simulink model "ASM_Traffic_MultiCore"  (R2026a)
settings: Solver=ode1  StartTime=SIM.tstart.v  StopTime=SIM.tend.v  FixedStep=SIM.StepSize.v
PostLoadFcn:
  | if any(exist('dsrtsu_mdlpostloadfcn', 'file') ~= 0), dsrtsu_mdlpostloadfcn('Execute', bdroot); end
  | try, asm_mdl_postloadfcn(bdroot, 'UpdateModel', 3600); catch, disp(lasterr); end,
InitFcn:
  | , if any(exist('rtifpga_mdlclblib', 'file') ~= 0), rtifpga_mdlclblib('Init', bdroot); end,
  | , if any(exist('dsmpb_private', 'file') ~= 0), dsmpb_private('dsmpb_mdlclblib', 'Init', bdroot); end,
model workspace (MAT data in the model file):
  asmReferencePath = [0 0.01 0.02 0.03 0.04 0.05 0.06 0.07 0.08 0.09 0.1 0.11 ... (350007 elements, 50001x7)]
  roadBounds : Simulink.Parameter (value not decoded)
  safetyAxes : Simulink.Parameter (value not decoded)
undefined symbols (not defined in the file): _to_, a0b2, ASM_BrakeHydraulics_DemoSystems, ASM_VehicleDynamics_DemoSystems, b98103fe8ad365046cd0, BrakeCircuit, controllerConfig, CPT, Crankshaft, DiscIntNeverNeededParam, dsmsi, FinalDriveAssembly, MDL, ModeSignals, mu, Pos_BrakePedal_Maneuver, rad, RefSignals, roadFamilyData, roadFamilyId, s_to_rpm, SIM, SoftECU, Suspension, Tire, Transmission
libraries: ASM_Traffic_lib x135, simulink x98, ASM_Utils_lib x77, ASM_VehicleDynamics_lib x70, ASM_Environment_lib x22, dsmpblib x20, dsmsilib x15, MDLD_Utils_lib x10, ASM_BrakeHydraulics_lib x3, sl_discontinuities x2
(part 30 of 65)

== system ASM_Traffic_MultiCore/Environment/SignalInterface/ExternalOutports/Select_Outport_Signals ==
  ASMSignalBus : Inport
  Bus Creator1 : BusCreator  Inputs=8
  Bus Creator2 : BusCreator  Inputs=8
  Bus Creator3 : BusCreator  Inputs=6
  Bus Creator4 : BusCreator  Inputs=5
  Bus Selector : BusSelector  OutputSignals=Maneuver,Road,Traffic,GroundTruth,Sensors
  Bus Selector1 : BusSelector  OutputSignals=Parameter,SensorIndex,Info,SensorOutput,SensorTimeStamp,RadarEffects,CustomPoints,ObjectData
  Bus Selector2 : BusSelector  OutputSignals=Parameter,SensorIndex,Info,SensorOutput,SensorTimeStamp,RadarEffects,CustomPoints,ObjectData
  Bus Selector3 : BusSelector  OutputSignals=Parameters,SensorIndex,SensorStatus,SensorOutput,Info,ObjectData
  Bus Selector4 : BusSelector  OutputSignals=Collision_Sensor,TrafficSign_Sensor_Dyn,Object_Sensor_3D.Sensor_1_Front_Long,Object_Sensor_3D.Sensor_2_Front_Mid,Object_Sensor_2D.Sensor_1_Front
  Maneuver : Outport  VectorParamsAs1DForOutWhenUnconnected=off
  Road : Outport  Port=2  VectorParamsAs1DForOutWhenUnconnected=off
  Traffic : Outport  Port=3  VectorParamsAs1DForOutWhenUnconnected=off
  GroundTruth : Outport  Port=4  VectorParamsAs1DForOutWhenUnconnected=off
  Sensors : Outport  Port=5  VectorParamsAs1DForOutWhenUnconnected=off
  wires:
  Bus Selector3/6 -> Bus Creator3/6  "<ObjectData>"
  Bus Selector3/5 -> Bus Creator3/5  "<Info>"
  Bus Selector3/4 -> Bus Creator3/4  "<SensorOutput>"
  Bus Selector3/3 -> Bus Creator3/3  "<SensorStatus>"
  Bus Selector3/2 -> Bus Creator3/2  "<SensorIndex>"
  Bus Selector3/1 -> Bus Creator3/1  "<Parameters>"
  Bus Creator3/1 -> Bus Creator4/5  "Object_Sensor_2D_1"
  Bus Selector4/5 -> Bus Selector3/1  "<Sensor_1_Front>"
  Bus Selector4/4 -> Bus Selector2/1  "<Sensor_2_Front_Mid>"
  Bus Selector2/1 -> Bus Creator2/1  "<Parameter>"
  Bus Selector2/2 -> Bus Creator2/2  "<SensorIndex>"
  Bus Selector2/3 -> Bus Creator2/3  "<Info>"
  Bus Selector2/4 -> Bus Creator2/4  "<SensorOutput>"
  Bus Selector2/5 -> Bus Creator2/5  "<SensorTimeStamp>"
  Bus Selector2/6 -> Bus Creator2/6  "<RadarEffects>"
  Bus Selector2/7 -> Bus Creator2/7  "<CustomPoints>"
  Bus Selector2/8 -> Bus Creator2/8  "<ObjectData>"
  Bus Creator2/1 -> Bus Creator4/4  "Object_Sensor_3D_2"
  Bus Creator1/1 -> Bus Creator4/3  "Object_Sensor_3D_1"
  Bus Selector1/8 -> Bus Creator1/8  "<ObjectData>"
  Bus Selector1/7 -> Bus Creator1/7  "<CustomPoints>"
  Bus Selector1/6 -> Bus Creator1/6  "<RadarEffects>"
  Bus Selector1/5 -> Bus Creator1/5  "<SensorTimeStamp>"
  Bus Selector1/4 -> Bus Creator1/4  "<SensorOutput>"
  Bus Selector1/3 -> Bus Creator1/3  "<Info>"
  Bus Selector1/2 -> Bus Creator1/2  "<SensorIndex>"
  Bus Selector1/1 -> Bus Creator1/1  "<Parameter>"
  Bus Selector4/3 -> Bus Selector1/1  "<Sensor_1_Front_Long>"
  Bus Selector4/2 -> Bus Creator4/2  "<TrafficSign_Sensor_Dyn>"
  Bus Selector/2 -> Road/1  "<Road>"
  Bus Selector/3 -> Traffic/1  "<Traffic>"
  Bus Selector/1 -> Maneuver/1  "<Maneuver>"
  ASMSignalBus/1 -> Bus Selector/1
  Bus Selector/4 -> GroundTruth/1  "<GroundTruth>"
  Bus Selector/5 -> Bus Selector4/1  "<Sensors>"
  Bus Selector4/1 -> Bus Creator4/1  "<Collision_Sensor>"
  Bus Creator4/1 -> Sensors/1  "Sensors"

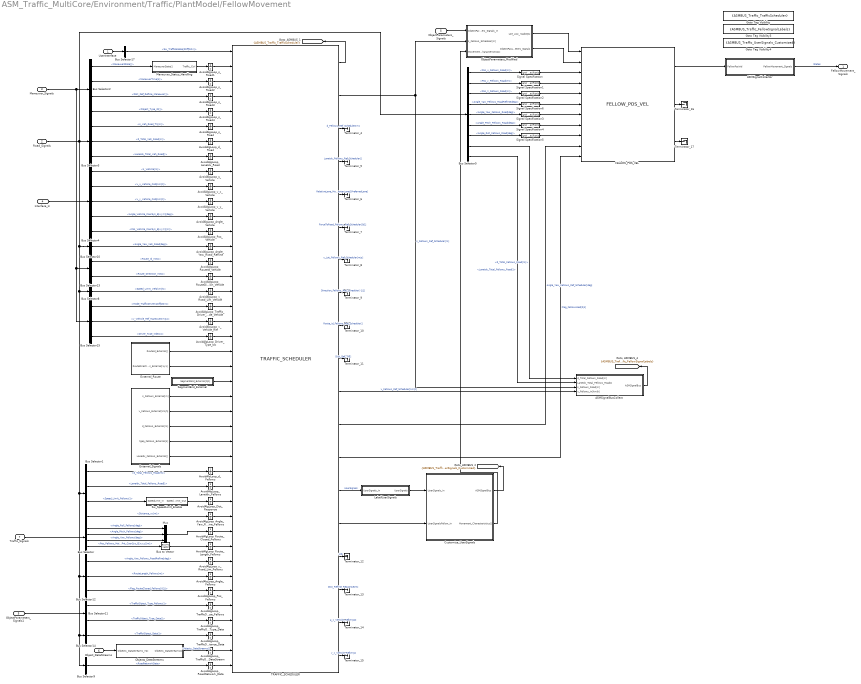
== system ASM_Traffic_MultiCore/Environment/Traffic/PlantModel/FellowMovement ==
  UserInterface : Inport
  Road_Signals : Inport  Port=2
  Maneuver_Signals : Inport  Port=3
  Interface_In : Inport  Port=4
  ObjectParameters_Signals : Inport  Port=5
  Object_DataStreams : Inport  Port=6
  Traffic_Signals : Inport  Port=7
  ASMSignalBusCollect : Subsystem
  ASMSignalCollector : Subsystem
  AvoidAlgLoop_Angle_Fellows : UnitDelay  SampleTime=-1
  AvoidAlgLoop_Angle_Vehicle : UnitDelay  SampleTime=-1
  AvoidAlgLoop_Angle_Yaw_RoadRefline_Fellows : UnitDelay  SampleTime=-1
  AvoidAlgLoop_Angle_Yaw_Road_Refline : UnitDelay  SampleTime=-1
  AvoidAlgLoop_Dist_Response : UnitDelay  SampleTime=-1
  AvoidAlgLoop_Driver_Type_Idx : UnitDelay  SampleTime=-1
  AvoidAlgLoop_LaneIdx_Fellows : UnitDelay  SampleTime=-1
  AvoidAlgLoop_LaneIdx_Road : UnitDelay  SampleTime=-1
  AvoidAlgLoop_Pos_Fellows : UnitDelay  SampleTime=-1
  AvoidAlgLoop_Pos_Vehicle : UnitDelay  SampleTime=-1
  AvoidAlgLoop_RoadNetwork_Data : UnitDelay  SampleTime=-1
  AvoidAlgLoop_RouteDirection_Vehicle : UnitDelay  SampleTime=-1
  AvoidAlgLoop_RouteId_Vehicle : UnitDelay  SampleTime=-1
  AvoidAlgLoop_Route_Closed_Fellows : UnitDelay  SampleTime=-1
  AvoidAlgLoop_Route_Length_Fellows : UnitDelay  SampleTime=-1
  AvoidAlgLoop_TrafficObject_DataStream : UnitDelay  SampleTime=-1
  AvoidAlgLoop_TrafficObject_Instance_Data : UnitDelay  SampleTime=-1
  AvoidAlgLoop_TrafficObject_Type_Data : UnitDelay  SampleTime=-1
  AvoidAlgLoop_TrafficObject_Type_Fellows : UnitDelay  SampleTime=-1
  AvoidAlgLoop_Traffic_Driver_Mode_Vehicle : UnitDelay  SampleTime=-1
  AvoidAlgLoop_d_Fellows : UnitDelay  SampleTime=-1
  AvoidAlgLoop_d_Road : UnitDelay  SampleTime=-1
  AvoidAlgLoop_s_Road{,1..4} (5 alike) : UnitDelay  SampleTime=-1
  AvoidAlgLoop_s_Vehicle : UnitDelay  SampleTime=-1
  AvoidAlgLoop_v_Road_Lim_Fellows : UnitDelay  SampleTime=-1
  AvoidAlgLoop_v_Road_Lim_Vehicle : UnitDelay  SampleTime=-1
  AvoidAlgLoop_v_Vehicle_Ref : UnitDelay  SampleTime=-1
  AvoidAlgLoop_v_x_Vehicle : UnitDelay  SampleTime=-1
  AvoidAlgLoop_v_y_Vehicle : UnitDelay  SampleTime=-1
  Bus Selector : BusSelector  OutputSignals=Plant.Traffic_Signals_toEnvironment.Angle_Fellows[x;y;z][deg].Angle_Roll_Fellows[deg],Plant.Traffic_Signals_toEnvironment.Angle_Fellows[x;y;z][deg].Angle_Pitch_Fellows[deg],Plant.Traffic_Signals_toEnvironment.Angle_Fellows[x;y;z][deg].Angle_Yaw_Fellows[deg],Plant.Traffic_Signals_toEnvironment.Pos_Fellows_MainPnt_CoorSys_E[x;y;z][m]
  Bus Selector1 : BusSelector  OutputSignals=Plant.Road_TrafficFellows.d_Total_Fellows_Road[m],Plant.Road_TrafficFellows.LaneIdx_Total_Fellows_Road[],Plant.Road_TrafficFellows.Speed_Limit_Fellows[],Plant.Road_TrafficFellows.Dist_Response_Traffic.Distance_xy[m]
  Bus Selector10 : BusSelector  OutputSignals=Plant.Road_ASMVeh.Angle_Yaw_Veh_Road[deg]
  Bus Selector11 : BusSelector  OutputSignals=FellowParameters.TrafficObject_Type_Fellows[],TrafficObjects.TrafficObject_Type_Data[]
  Bus Selector12 : BusSelector  OutputSignals=Plant.Road_TrafficFellows.Angle_Yaw_Fellows_RoadRefline[deg],Plant.Road_TrafficFellows.RouteLength_Fellows[m],Plant.Road_TrafficFellows.Flag_RouteClosed_Fellows[0|1]
  Bus Selector13 : BusSelector  OutputSignals=Plant.ManeuverScheduler.InitialVehStates.Route_Id_Init[],Plant.ManeuverScheduler.InitialVehStates.Route_Direction_Init[]
  Bus Selector14 : BusSelector  OutputSignals=Plant.TrafficObject_Data[]
  Bus Selector15 : BusSelector  OutputSignals=Plant.ManeuverScheduler.ModeSignals.Mode_TrafficDriver[1Off|2On],Plant.ManeuverScheduler.RefSignals.v_Vehicle_Ref_Maneuver[m|s],Plant.ManeuverScheduler.Parameters.Driver_Type_Index[]
  Bus Selector17 : BusSelector  OutputSignals=Sw_TrafficEnable[0Off|1On]
  Bus Selector2 : BusSelector  OutputSignals=Plant.ManeuverScheduler.Info.ManeuverState[],Plant.ManeuverScheduler.Info.ManeuverTime[s],Plant.ManeuverScheduler.RefSignals.Dist_Def_Refline_Maneuver[],Plant.ManeuverScheduler.Parameters.Object_Type_ID[]
  Bus Selector3 : BusSelector  OutputSignals=Plant.Road_ASMVeh.s_Veh_Road_Trj[m],Plant.Road_ASMVeh.d_Total_Veh_Road[m],Plant.Road_ASMVeh.LaneIdx_Total_Veh_Road[]
  Bus Selector4 : BusSelector  OutputSignals=ExternalModel.s_Vehicle[m],ExternalModel.v_x_Vehicle_CoG[km|h],ExternalModel.v_y_Vehicle_CoG[km|h],ExternalModel.Angle_Vehicle_CoorSys_E[x;y;z][deg],ExternalModel.Pos_Vehicle_CoorSys_E[x;y;z][m]
  Bus Selector5 : BusSelector  OutputSignals=Plant.Road_TrafficFellows.Pos_x_Fellows_Road[m],Plant.Road_TrafficFellows.Pos_y_Fellows_Road[m],Plant.Road_TrafficFellows.Pos_z_Fellows_Road[m],Plant.Road_TrafficFellows.Angle_Yaw_Fellows_RoadRefline[deg],Plant.Road_TrafficFellows.Angle_Yaw_Fellows_Road[deg],Plant.Road_TrafficFellows.Angle_Pitch_Fellows_Road[deg],Plant.Road_TrafficFellows.Angle_Roll_Fellows_Road[deg],Plant.Road_TrafficFellows.d_Total_Fellows_Road[m],Plant.Road_TrafficFellows.LaneIdx_Total_Fellows_Road[]
  Bus Selector8 : BusSelector  OutputSignals=Plant.Road_Info.Speed_Limit_Veh[km|h]
  Bus Selector9 : BusSelector  OutputSignals=Plant.Road_Info.Trf_Driver_Data.RoadNetworkData
  Bus to Vector : BusToVector
  Customize_UserSignals : Subsystem
  External_Route : Subsystem
  External_Signals : Subsystem
  FELLOW_POS_VEL : ASM_Traffic_lib/Movement/FELLOW_POS_VEL  StepSize=SIM.StepSize  ASMProperties=struct('Name','FELLOW_POS_VEL','Version','2.0','Library','ASM_Traffic_lib')  ASMInstanceName=fellow_pos_vel  ASMInstanceID=1
  Goto Tag Visibility : GotoTagVisibility  GotoTag=ASMBUS_Traffic_TrafficScheduler
  Goto Tag Visibility3 : GotoTagVisibility  GotoTag=ASMBUS_Traffic_FellowSignalLabels
  Goto Tag Visibility4 : GotoTagVisibility  GotoTag=ASMBUS_Traffic_UserSignals_Customized
  LabelUserSignals : Subsystem
  Maneuver_Status_Handling : Subsystem
  Mux : Mux  Inputs=3
  ObjectParameters_Modified : Subsystem
  ObjectParameters_Signals1 : InportShadow  Port=5
  Objects_DataStreams : Subsystem
  SegmentEnd_External : Subsystem
  Signal Specification{,1..6} (7 alike) : SignalSpecification  Dimensions=MDL.Traffic.MaxNumFellows.v
  Sw_SpeedLimit_Enable : Subsystem
  TRAFFIC_SCHEDULER : ASM_Traffic_lib/Movement/TRAFFIC_SCHEDULER  Tag=ASM_SUBCOMPONENT  TrafficVector=MDL.Traffic.TrafficScheduler.Scenario  MaxNumFellows=MDL.Traffic.MaxNumFellows  MaxNumFDUserSignals=MDL.Traffic.MaxNumFDUserSignals  MaxNumUserSignals=MDL.Traffic.MaxNumUserSignals  StepSize=SIM.StepSize  ASMProperties=struct('Name','TRAFFIC_SCHEDULER','Version','23.0','Library','ASM_Traffic_lib')  ASMInstanceName=traffic_scheduler  ASMInstanceID=1
  Terminator_{4..17} (14 alike) : Terminator
  FellowMovement_Signals : Outport  VectorParamsAs1DForOutWhenUnconnected=off
  tag scope: ASMBUS_Traffic_FellowSignalLabels=scoped, ASMBUS_Traffic_TrafficScheduler=scoped, ASMBUS_Traffic_UserSignals_Customized=scoped
  wires:
  ObjectParameters_Modified/2(ObjectParameters_Signals) -> FELLOW_POS_VEL/2
  FELLOW_POS_VEL/1 -> ASMSignalCollector/1(FellowPosVel)
  TRAFFIC_SCHEDULER/19 -> Terminator_15/1  "v_x_Vehicle_Ref[m|s]"
  TRAFFIC_SCHEDULER/18 -> Terminator_14/1  "a_x_Vehicle_Ref[m|s2]"
  TRAFFIC_SCHEDULER/17 -> Terminator_13/1  "Dist_Refline_Response[m]"
  TRAFFIC_SCHEDULER/16 -> Terminator_12/1  "Info"
  TRAFFIC_SCHEDULER/10 -> Terminator_11/1  "Dist_Def_Trf[]"
  TRAFFIC_SCHEDULER/9 -> Terminator_10/1  "Route_Id_Fellows_Ref_Scheduler[]"
  TRAFFIC_SCHEDULER/8 -> Terminator_9/1  "Direction_Fellows_Ref_Scheduler[-1|1]"
  TRAFFIC_SCHEDULER/7 -> Terminator_8/1  "v_Lat_Fellows_Ref_Scheduler[m|s]"
  TRAFFIC_SCHEDULER/6 -> Terminator_7/1  "ForceToRoad_Fellows_Ref_Scheduler[0|1]"
  TRAFFIC_SCHEDULER/5 -> Terminator_6/1  "RelativeLane_Mode_Fellows[0CenterLane|1PreferredLane]"
  TRAFFIC_SCHEDULER/4 -> Terminator_5/1  "LaneIdx_Fellows_Ref_Scheduler[]"
  TRAFFIC_SCHEDULER/3 -> Terminator_4/1  "d_Fellows_Ref_Scheduler[m]"
  Customize_UserSignals/2(Movement_Characteristics[]) -> ObjectParameters_Modified/3(Movement_Characteristics[])
  ASMSignalCollector/1(FellowMovement_Signals) -> FellowMovement_Signals/1  "States"
  Object_DataStreams/1 -> Objects_DataStreams/1(Objects_DataStreams_In[])
  Bus Selector17/1 -> TRAFFIC_SCHEDULER/1  "<Sw_TrafficEnable[0Off|1On]>"
  UserInterface/1 -> Bus Selector17/1
  TRAFFIC_SCHEDULER/11 -> ASMSignalBusCollect/4(v_Fellows_In[km|h])  "v_Fellows_Ref_Scheduler[km|h]"
  TRAFFIC_SCHEDULER/12 -> FELLOW_POS_VEL/10  "Angle_Yaw_Fellows_Ref_Scheduler[deg]"
  TRAFFIC_SCHEDULER/13 -> FELLOW_POS_VEL/11  "Flag_FellowUsed[0|1]"
  TRAFFIC_SCHEDULER/14 -> LabelUserSignals/1(UserSignals_In)  "UserSignals"
  TRAFFIC_SCHEDULER/15 -> Customize_UserSignals/2(UserSignalsFellow_In)
  Bus Selector12/3 -> AvoidAlgLoop_Pos_Fellows/1  "<Flag_RouteClosed_Fellows[0|1]>"
  Bus Selector12/2 -> AvoidAlgLoop_Angle_Fellows/1  "<RouteLength_Fellows[m]>"
  Bus Selector12/1 -> AvoidAlgLoop_v_Road_Lim_Fellows/1  "<Angle_Yaw_Fellows_RoadRefline[deg]>"
  Bus Selector1/3 -> Sw_SpeedLimit_Enable/1(SpeedLimit_In)  "<Speed_Limit_Fellows[]>"
  Sw_SpeedLimit_Enable/1(SpeedLimit_Out) -> AvoidAlgLoop_Dist_Response/1
  AvoidAlgLoop_TrafficObject_DataStream/1 -> TRAFFIC_SCHEDULER/41
  Objects_DataStreams/1(Objects_DataStreams[]) -> AvoidAlgLoop_TrafficObject_DataStream/1  "Objects_DataStreams[]"
  AvoidAlgLoop_RoadNetwork_Data/1 -> TRAFFIC_SCHEDULER/42
  Bus Selector8/1 -> AvoidAlgLoop_v_Road_Lim_Vehicle/1  "<Speed_Limit_Veh[km|h]>"
  Bus Selector4/5 -> AvoidAlgLoop_Pos_Vehicle/1  "<Pos_Vehicle_CoorSys_E[x;y;z][m]>"
  Bus Selector4/4 -> AvoidAlgLoop_Angle_Vehicle/1  "<Angle_Vehicle_CoorSys_E[x;y;z][deg]>"
  AvoidAlgLoop_Angle_Vehicle/1 -> TRAFFIC_SCHEDULER/12
  AvoidAlgLoop_Pos_Fellows/1 -> TRAFFIC_SCHEDULER/37
  AvoidAlgLoop_v_Road_Lim_Vehicle/1 -> TRAFFIC_SCHEDULER/17
  Bus Selector15/3 -> AvoidAlgLoop_Driver_Type_Idx/1  "<Driver_Type_Index[]>"
  Bus Selector15/1 -> AvoidAlgLoop_Traffic_Driver_Mode_Vehicle/1  "<Mode_TrafficDriver[1Off|2On]>"
  AvoidAlgLoop_Traffic_Driver_Mode_Vehicle/1 -> TRAFFIC_SCHEDULER/18
  AvoidAlgLoop_Driver_Type_Idx/1 -> TRAFFIC_SCHEDULER/20
  AvoidAlgLoop_v_Vehicle_Ref/1 -> TRAFFIC_SCHEDULER/19
  Bus Selector15/2 -> AvoidAlgLoop_v_Vehicle_Ref/1  "<v_Vehicle_Ref_Maneuver[m|s]>"
  AvoidAlgLoop_v_y_Vehicle/1 -> TRAFFIC_SCHEDULER/11
  AvoidAlgLoop_Pos_Vehicle/1 -> TRAFFIC_SCHEDULER/13
  Maneuver_Signals/1 -> Bus Selector13/1, Bus Selector15/1, Bus Selector2/1
  AvoidAlgLoop_LaneIdx_Fellows/1 -> TRAFFIC_SCHEDULER/30
  AvoidAlgLoop_v_Road_Lim_Fellows/1 -> TRAFFIC_SCHEDULER/35
  AvoidAlgLoop_Angle_Yaw_RoadRefline_Fellows/1 -> TRAFFIC_SCHEDULER/32
  Bus Selector14/1 -> AvoidAlgLoop_TrafficObject_Instance_Data/1  "<TrafficObject_Data[]>"
  Bus Selector9/1 -> AvoidAlgLoop_RoadNetwork_Data/1  "<RoadNetworkData>"
  AvoidAlgLoop_s_Road3/1 -> TRAFFIC_SCHEDULER/4
  AvoidAlgLoop_s_Road/1 -> TRAFFIC_SCHEDULER/6
  AvoidAlgLoop_RouteDirection_Vehicle/1 -> TRAFFIC_SCHEDULER/16
  TRAFFIC_SCHEDULER/1 -> [ASMBUS_Traffic_TrafficScheduler]
  AvoidAlgLoop_s_Road2/1 -> TRAFFIC_SCHEDULER/3
  External_Signals/3(d_Fellows_External[m]) -> TRAFFIC_SCHEDULER/26
  External_Signals/1(s_Fellows_External[m]) -> TRAFFIC_SCHEDULER/24
  AvoidAlgLoop_TrafficObject_Type_Data/1 -> TRAFFIC_SCHEDULER/39
  AvoidAlgLoop_v_x_Vehicle/1 -> TRAFFIC_SCHEDULER/10
  AvoidAlgLoop_TrafficObject_Type_Fellows/1 -> TRAFFIC_SCHEDULER/38
  External_Signals/2(v_Fellows_External[km|h]) -> TRAFFIC_SCHEDULER/25
  AvoidAlgLoop_s_Road4/1 -> TRAFFIC_SCHEDULER/5
  Bus Selector13/1 -> AvoidAlgLoop_RouteId_Vehicle/1  "<Route_Id_Init[]>"
  AvoidAlgLoop_Angle_Fellows/1 -> TRAFFIC_SCHEDULER/36
  AvoidAlgLoop_s_Vehicle/1 -> TRAFFIC_SCHEDULER/9
  AvoidAlgLoop_d_Fellows/1 -> TRAFFIC_SCHEDULER/29
  Bus Selector4/1 -> AvoidAlgLoop_s_Vehicle/1  "<s_Vehicle[m]>"
  Bus Selector11/1 -> AvoidAlgLoop_TrafficObject_Type_Fellows/1  "<TrafficObject_Type_Fellows[]>"
  AvoidAlgLoop_TrafficObject_Instance_Data/1 -> TRAFFIC_SCHEDULER/40
  Bus Selector2/4 -> AvoidAlgLoop_s_Road4/1  "<Object_Type_ID[]>"
  Bus Selector3/3 -> AvoidAlgLoop_LaneIdx_Road/1  "<LaneIdx_Total_Veh_Road[]>"
  Interface_In/1 -> Bus Selector4/1
  Bus Selector3/1 -> AvoidAlgLoop_s_Road/1  "<s_Veh_Road_Trj[m]>"
  Bus Selector4/3 -> AvoidAlgLoop_v_y_Vehicle/1  "<v_y_Vehicle_CoG[km|h]>"
  Maneuver_Status_Handling/1(Traffic_Ctrl) -> AvoidAlgLoop_s_Road1/1
  Bus Selector1/1 -> AvoidAlgLoop_d_Fellows/1  "<d_Total_Fellows_Road[m]>"
  Bus Selector1/2 -> AvoidAlgLoop_LaneIdx_Fellows/1  "<LaneIdx_Total_Fellows_Road[]>"
  Bus Selector3/2 -> AvoidAlgLoop_d_Road/1  "<d_Total_Veh_Road[m]>"
  Bus Selector2/1 -> Maneuver_Status_Handling/1(ManeuverState[])  "<ManeuverState[]>"
  Bus Selector4/2 -> AvoidAlgLoop_v_x_Vehicle/1  "<v_x_Vehicle_CoG[km|h]>"
  TRAFFIC_SCHEDULER/2 -> ObjectParameters_Modified/2(s_Fellows_Scheduler[m]), ASMSignalBusCollect/3(s_Fellows_Road[m])  "s_Fellows_Ref_Scheduler[m]"
  AvoidAlgLoop_LaneIdx_Road/1 -> TRAFFIC_SCHEDULER/8
  Bus Selector2/2 -> AvoidAlgLoop_s_Road2/1  "<ManeuverTime[s]>"
  AvoidAlgLoop_Dist_Response/1 -> TRAFFIC_SCHEDULER/31
  LabelUserSignals/1(UserSignals) -> Customize_UserSignals/1(UserSignals_In)
  Road_Signals/1 -> Bus Selector3/1, Bus Selector10/1, Bus Selector1/1, Bus Selector12/1, Bus Selector14/1, Bus Selector9/1, Bus Selector8/1, Bus Selector5/1
  Bus Selector2/3 -> AvoidAlgLoop_s_Road3/1  "<Dist_Def_Refline_Maneuver[]>"
  AvoidAlgLoop_d_Road/1 -> TRAFFIC_SCHEDULER/7
  ObjectParameters_Signals1/1 -> Bus Selector11/1
  Bus Selector10/1 -> AvoidAlgLoop_Angle_Yaw_Road_Refline/1  "<Angle_Yaw_Veh_Road[deg]>"
  AvoidAlgLoop_RouteId_Vehicle/1 -> TRAFFIC_SCHEDULER/15
  AvoidAlgLoop_s_Road1/1 -> TRAFFIC_SCHEDULER/2
  External_Route/1(RouteId_External[]) -> TRAFFIC_SCHEDULER/21
  Bus Selector11/2 -> AvoidAlgLoop_TrafficObject_Type_Data/1  "<TrafficObject_Type_Data[]>"
  External_Signals/4(tgap_Fellows_External[s]) -> TRAFFIC_SCHEDULER/27
  SegmentEnd_External/1(SegmentEnd_External[0|1]) -> TRAFFIC_SCHEDULER/23
  AvoidAlgLoop_Angle_Yaw_Road_Refline/1 -> TRAFFIC_SCHEDULER/14
  Bus Selector1/4 -> AvoidAlgLoop_Angle_Yaw_RoadRefline_Fellows/1  "<Distance_xy[m]>"
  Bus Selector13/2 -> AvoidAlgLoop_RouteDirection_Vehicle/1  "<Route_Direction_Init[]>"
  External_Signals/5(LaneIdx_Fellows_External[]) -> TRAFFIC_SCHEDULER/28
  External_Route/2(RouteDirection_External[1|-1]) -> TRAFFIC_SCHEDULER/22
  ASMSignalBusCollect/1(ASMSignalBus) -> [ASMBUS_Traffic_FellowSignalLabels]
  Bus Selector5/9 -> ASMSignalBusCollect/2(LaneIdx_Total_Fellows_Road[])  "<LaneIdx_Total_Fellows_Road[]>"
  Bus Selector5/8 -> ASMSignalBusCollect/1(d_Total_Fellows_Road[m])  "<d_Total_Fellows_Road[m]>"
  Customize_UserSignals/1(ASMSignalBus) -> [ASMBUS_Traffic_UserSignals_Customized]
  ObjectParameters_Signals/1 -> ObjectParameters_Modified/1(ObjectParameters_Signals_In)
  Bus Selector5/7 -> Signal Specification5/1  "<Angle_Roll_Fellows_Road[deg]>"
  Bus Selector5/6 -> Signal Specification4/1  "<Angle_Pitch_Fellows_Road[deg]>"
  Bus Selector5/5 -> Signal Specification3/1  "<Angle_Yaw_Fellows_Road[deg]>"
  Bus Selector5/3 -> Signal Specification2/1  "<Pos_z_Fellows_Road[m]>"
  Bus Selector5/2 -> Signal Specification1/1  "<Pos_y_Fellows_Road[m]>"
  Bus Selector5/1 -> Signal Specification/1  "<Pos_x_Fellows_Road[m]>"
  Signal Specification/1 -> FELLOW_POS_VEL/3
  Signal Specification1/1 -> FELLOW_POS_VEL/4
  Signal Specification2/1 -> FELLOW_POS_VEL/5
  Signal Specification4/1 -> FELLOW_POS_VEL/8
  Signal Specification5/1 -> FELLOW_POS_VEL/9
  FELLOW_POS_VEL/2 -> Terminator_16/1
  FELLOW_POS_VEL/3 -> Terminator_17/1
  Traffic_Signals/1 -> Bus Selector/1
  Bus Selector/4 -> Bus to Vector/1  "<Pos_Fellows_MainPnt_CoorSys_E[x;y;z][m]>"
  Bus to Vector/1 -> AvoidAlgLoop_Route_Length_Fellows/1
  Mux/1 -> AvoidAlgLoop_Route_Closed_Fellows/1
  Bus Selector/1 -> Mux/1  "<Angle_Roll_Fellows[deg]>"
  Bus Selector/2 -> Mux/2  "<Angle_Pitch_Fellows[deg]>"
  Bus Selector/3 -> Mux/3  "<Angle_Yaw_Fellows[deg]>"
  AvoidAlgLoop_Route_Closed_Fellows/1 -> TRAFFIC_SCHEDULER/33
  AvoidAlgLoop_Route_Length_Fellows/1 -> TRAFFIC_SCHEDULER/34
  Bus Selector5/4 -> Signal Specification6/1  "<Angle_Yaw_Fellows_RoadRefline[deg]>"
  Signal Specification3/1 -> FELLOW_POS_VEL/7
  Signal Specification6/1 -> FELLOW_POS_VEL/6
  ObjectParameters_Modified/1(use_yaw_road[0|1]) -> FELLOW_POS_VEL/1

== system ASM_Traffic_MultiCore/Environment/Traffic/PlantModel/Merge_Signals_toEnvironment ==
  Traffic_Signals : Inport
  GroundTruth_Interface : Inport  Port=2
  Bus Creator : BusCreator  Inputs=26
  Bus Selector : BusSelector  OutputSignals=TrafficScheduler
  Bus Selector1 : BusSelector  OutputSignals=Plant.Control
  Bus Selector2 : BusSelector  OutputSignals=s_Fellows_Ref_Scheduler[m],d_Fellows_Ref_Scheduler[m],v_Fellows_Ref_Scheduler[km|h],LaneIdx_Fellows_Ref_Scheduler[],RelativeLane_Mode_Fellows[0CenterLane|1PreferredLane],ForceToRoad_Fellows_Ref_Scheduler[0|1],v_Lat_Fellows_Ref_Scheduler[m|s],Direction_Fellows_Ref_Scheduler[-1|1],Route_Id_Fellows_Ref_Scheduler[],Dist_Def_Trf[],Flag_FellowUsed[0|1],a_x_Vehicle_Ref[m|s2],Dist_Refline_Response[m],Info,a_Fellows_Ref_Scheduler[m|s2],UserSignals_Fellows[]
  Bus Selector3 : BusSelector  OutputSignals=FellowPositions
  Bus Selector4 : BusSelector  OutputSignals=FellowSignalLabels
  Bus Selector5 : BusSelector  OutputSignals=d_Total_Fellows[m],LaneIdx_Total_Fellows[],v_Fellows[km|h]
  Bus Selector6 : BusSelector  OutputSignals=Pos_Fellows_MainPnt_CoorSys_E[x;y;z][m],Angle_Fellows[x;y;z][deg],Angle_Fellows[x;y;z][deg].Angle_Wheel_Fellows[deg]
  Bus Selector7 : BusSelector  OutputSignals=FellowVelocities
  Bus Selector8 : BusSelector  OutputSignals=v_Fellows[x;y;z][km|h],w_Fellows[x;y;z][deg|s]
  Bus Selector9 : BusSelector  OutputSignals=UserSignals_Customized
  avoid_incomplete_trace2source : Subsystem
  Signals_toEnvironment : Outport  VectorParamsAs1DForOutWhenUnconnected=off
  wires:
  avoid_incomplete_trace2source/1(Out1) -> Bus Creator/26  "Control"
  Bus Selector1/1 -> avoid_incomplete_trace2source/1(In1)  "<Control>"
  Bus Selector9/1 -> Bus Creator/25  "<UserSignals_Customized>"
  Bus Selector8/2 -> Bus Creator/24  "<w_Fellows[x;y;z][deg|s]>"
  Bus Selector8/1 -> Bus Creator/23  "<v_Fellows[x;y;z][km|h]>"
  Bus Selector6/3 -> Bus Creator/22  "<Angle_Wheel_Fellows[deg]>"
  Bus Selector6/2 -> Bus Creator/21  "<Angle_Fellows[x;y;z][deg]>"
  Bus Selector6/1 -> Bus Creator/20  "<Pos_Fellows_MainPnt_CoorSys_E[x;y;z][m]>"
  Bus Selector5/3 -> Bus Creator/19  "<v_Fellows[km|h]>"
  Bus Selector5/2 -> Bus Creator/18  "<LaneIdx_Total_Fellows[]>"
  Bus Selector5/1 -> Bus Creator/17  "<d_Total_Fellows[m]>"
  Bus Selector2/16 -> Bus Creator/16  "<UserSignals_Fellows[]>"
  Bus Selector2/15 -> Bus Creator/15  "<a_Fellows_Ref_Scheduler[m|s2]>"
  Bus Selector2/14 -> Bus Creator/14  "<Info>"
  Bus Selector2/13 -> Bus Creator/13  "<Dist_Refline_Response[m]>"
  Bus Selector7/1 -> Bus Selector8/1  "<FellowVelocities>"
  Bus Selector3/1 -> Bus Selector6/1  "<FellowPositions>"
  Bus Selector4/1 -> Bus Selector5/1  "<FellowSignalLabels>"
  Traffic_Signals/1 -> Bus Selector/1, Bus Selector7/1, Bus Selector9/1, Bus Selector3/1, Bus Selector4/1
  Bus Selector/1 -> Bus Selector2/1  "<TrafficScheduler>"
  Bus Selector2/12 -> Bus Creator/12  "<a_x_Vehicle_Ref[m|s2]>"
  GroundTruth_Interface/1 -> Bus Selector1/1
  Bus Selector2/2 -> Bus Creator/2  "<d_Fellows_Ref_Scheduler[m]>"
  Bus Selector2/1 -> Bus Creator/1  "<s_Fellows_Ref_Scheduler[m]>"
  Bus Selector2/4 -> Bus Creator/4  "<LaneIdx_Fellows_Ref_Scheduler[]>"
  Bus Selector2/5 -> Bus Creator/5  "<RelativeLane_Mode_Fellows[0CenterLane|1PreferredLane]>"
  Bus Selector2/6 -> Bus Creator/6  "<ForceToRoad_Fellows_Ref_Scheduler[0|1]>"
  Bus Selector2/7 -> Bus Creator/7  "<v_Lat_Fellows_Ref_Scheduler[m|s]>"
  Bus Selector2/8 -> Bus Creator/8  "<Direction_Fellows_Ref_Scheduler[-1|1]>"
  Bus Selector2/9 -> Bus Creator/9  "<Route_Id_Fellows_Ref_Scheduler[]>"
  Bus Selector2/10 -> Bus Creator/10  "<Dist_Def_Trf[]>"
  Bus Selector2/11 -> Bus Creator/11  "<Flag_FellowUsed[0|1]>"
  Bus Creator/1 -> Signals_toEnvironment/1  "Traffic_Signals_toEnvironment"
  Bus Selector2/3 -> Bus Creator/3  "<v_Fellows_Ref_Scheduler[km|h]>"

== system ASM_Traffic_MultiCore/Environment/Traffic/PlantModel/ObjectParameters ==
  Road_Signals : Inport
  Maneuver_Signals : Inport  Port=2
  Sensor_Signals : Inport  Port=3
  ASMSignalCollector : Subsystem
  Bus Creator1 : BusCreator  Inputs=7
  Bus Selector : BusSelector  OutputSignals=UserInterface.Sw_RoadSelect[1_6],Plant.Road_Info.RoadState[]
  Bus Selector1 : BusSelector  OutputSignals=TrafficObjects.Flag_TrafficObject_Init_Ready[0|1]
  Bus Selector2 : BusSelector  OutputSignals=Plant.ManeuverScheduler.MdlControl.RoadControl[]
  Bus Selector3 : BusSelector  OutputSignals=Plant.Object_Sensor_2D.Sensors_2D_Common.Sw_Enable_Discrete_Objects[0Off|1On]
  DISCRETE_OBJECTS : ASM_Traffic_lib/Objects/DISCRETE_OBJECTS  Tag=ASM_SUBCOMPONENT  DiscreteObjects_1=MDL.Traffic.DiscreteObjects.DiscreteObjects_1  DiscreteObjects_2=MDL.Traffic.DiscreteObjects.DiscreteObjects_2  DiscreteObjects_3=MDL.Traffic.DiscreteObjects.DiscreteObjects_3  DiscreteObjects_4=MDL.Traffic.DiscreteObjects.DiscreteObjects_4  DiscreteObjects_5=MDL.Traffic.DiscreteObjects.DiscreteObjects_5  DiscreteObjects_6=MDL.Traffic.DiscreteObjects.DiscreteObjects_6  Const_Length_Bounding_Rectangle_Quadrant=MDL.Traffic.DiscreteObjects.Const_Length_Bounding_Rectangle_Quadrant  ASMProperties=struct('Name','DISCRETE_OBJECTS','Version','9.0','Library','ASM_Traffic_lib')  ASMInstanceName=discrete_objects  ASMInstanceID=1
  FELLOW_PARAMETERS : ASM_Traffic_lib/Objects/FELLOW_PARAMETERS  Tag=ASM_SUBCOMPONENT  TrafficObject_Type_Fellows=MDL.Traffic.Sensors.Fellows.TrafficObject_Type_Fellows  MaxNumFellows=MDL.Traffic.MaxNumFellows.v  ASMProperties=struct('Name','FELLOW_PARAMETERS','Version','13.0','Library','ASM_Traffic_lib')  ASMInstanceName=fellow_parameters  ASMInstanceID=1
  Goto Tag Visibility : GotoTagVisibility  GotoTag=ASMBUS_Environment_Traffic_TrafficObjects
  Goto Tag Visibility1 : GotoTagVisibility  GotoTag=ASMBUS_Environment_Traffic_FellowParameters
  Goto Tag Visibility2 : GotoTagVisibility  GotoTag=ASMBUS_Environment_Traffic_DiscreteObjects
  TRAFFIC_OBJECTS : ASM_Traffic_lib/Objects/TRAFFIC_OBJECTS  Tag=ASM_SUBCOMPONENT  ObjRoad_1=MDL.Traffic.Objects.RoadObjects_1  ObjRoad_2=MDL.Traffic.Objects.RoadObjects_2  ObjRoad_3=MDL.Traffic.Objects.RoadObjects_3  ObjRoad_4=MDL.Traffic.Objects.RoadObjects_4  ObjRoad_5=MDL.Traffic.Objects.RoadObjects_5  ObjRoad_6=MDL.Traffic.Objects.RoadObjects_6  ObjTraffic=MDL.Traffic.Objects.TrafficObjects  ASMProperties=struct('Name','TRAFFIC_OBJECTS','Version','7.0','Library','ASM_Traffic_lib')  ASMInstanceName=traffic_objects  ASMInstanceID=1
  Terminator : Terminator
  Terminator1 : Terminator
  Terminator2 : Terminator
  TrafficObject_Reload_Trigger : Subsystem
  Objects_Signals : Outport  VectorParamsAs1DForOutWhenUnconnected=off
  tag scope: ASMBUS_Environment_Traffic_DiscreteObjects=scoped, ASMBUS_Environment_Traffic_FellowParameters=scoped, ASMBUS_Environment_Traffic_TrafficObjects=scoped
  wires:
  Bus Selector2/1 -> TrafficObject_Reload_Trigger/2(RoadControl[])  "<RoadControl[]>"
  Maneuver_Signals/1 -> Bus Selector2/1
  Bus Selector/1 -> DISCRETE_OBJECTS/1, TRAFFIC_OBJECTS/1  "<Sw_RoadSelect[1_6]>"
  ASMSignalCollector/1(ObjectParameter_Signals) -> Bus Selector1/1, Objects_Signals/1
  TrafficObject_Reload_Trigger/1(Ctrl) -> TRAFFIC_OBJECTS/2
  DISCRETE_OBJECTS/2 -> Terminator/1  "DiscreteObject_Data[]"
  DISCRETE_OBJECTS/1 -> [ASMBUS_Environment_Traffic_DiscreteObjects]
  FELLOW_PARAMETERS/9 -> Terminator1/1  "TrafficObject_Type_Fellows[]"
  FELLOW_PARAMETERS/2 -> Bus Creator1/1
  TRAFFIC_OBJECTS/1 -> [ASMBUS_Environment_Traffic_TrafficObjects]
  Bus Selector/2 -> TrafficObject_Reload_Trigger/1(RoadState[])  "<RoadState[]>"
  Road_Signals/1 -> Bus Selector/1
  TRAFFIC_OBJECTS/2 -> FELLOW_PARAMETERS/1  "TrafficObject_Type_Data[]"
  FELLOW_PARAMETERS/5 -> Bus Creator1/4
  FELLOW_PARAMETERS/4 -> Bus Creator1/3
  FELLOW_PARAMETERS/1 -> [ASMBUS_Environment_Traffic_FellowParameters]
  FELLOW_PARAMETERS/8 -> Bus Creator1/7
  FELLOW_PARAMETERS/7 -> Bus Creator1/6
  FELLOW_PARAMETERS/6 -> Bus Creator1/5
  FELLOW_PARAMETERS/3 -> Bus Creator1/2
  Bus Selector1/1 -> DISCRETE_OBJECTS/3  "<Flag_TrafficObject_Init_Ready[0|1]>"
  Bus Creator1/1 -> Terminator2/1  "FellowsGeometry"
  Sensor_Signals/1 -> Bus Selector3/1
  Bus Selector3/1 -> DISCRETE_OBJECTS/2  "<Sw_Enable_Discrete_Objects[0Off|1On]>"

== system ASM_Traffic_MultiCore/Environment/Traffic/PlantModel/V2X ==
  Road_Signals : Inport
  Maneuver_Signals : Inport  Port=2
  UserInterface : Inport  Port=3
  ASMSignalCollector : Subsystem
  Bus Selector : BusSelector  OutputSignals=Plant.ManeuverScheduler.Info.ManeuverTime[s]
  Bus Selector1 : BusSelector  OutputSignals=Plant.Road_Info.RoadState[],Plant.Road_Info.V2X_Data[]
  Bus Selector2 : BusSelector  OutputSignals=V2X.Reset[0|1]
  Goto Tag Visibility : GotoTagVisibility  GotoTag=ASMBUS_Traffic_V2X_TrafficLightController
  V2X_TRAFFIC_LIGHT_CONTROLLER : ASM_Traffic_lib/SoftECU/V2X_TRAFFIC_LIGHT_CONTROLLER  Tag=ASM_SUBCOMPONENT  ASMProperties=struct('Name','V2X_TRAFFIC_LIGHT_CONTROLLER','Version','2.0','Library','ASM_Traffic_lib')  ASMInstanceName=v2x_traffic_light_controller  ASMInstanceID=1
  V2X_Signals : Outport  VectorParamsAs1DForOutWhenUnconnected=off
  tag scope: ASMBUS_Traffic_V2X_TrafficLightController=scoped
  wires:
  Maneuver_Signals/1 -> Bus Selector/1
  Bus Selector/1 -> V2X_TRAFFIC_LIGHT_CONTROLLER/2  "<ManeuverTime[s]>"
  Road_Signals/1 -> Bus Selector1/1
  Bus Selector1/1 -> V2X_TRAFFIC_LIGHT_CONTROLLER/3  "<RoadState[]>"
  Bus Selector1/2 -> V2X_TRAFFIC_LIGHT_CONTROLLER/4  "<V2X_Data[]>"
  V2X_TRAFFIC_LIGHT_CONTROLLER/1 -> [ASMBUS_Traffic_V2X_TrafficLightController]
  ASMSignalCollector/1(V2X_Signals) -> V2X_Signals/1
  UserInterface/1 -> Bus Selector2/1
  Bus Selector2/1 -> V2X_TRAFFIC_LIGHT_CONTROLLER/1  "<Reset[0|1]>"

== system ASM_Traffic_MultiCore/Environment/Traffic/UserInterface/ASMSignalBus_Plant ==
  In : Inport
  Terminator_2 : Terminator
  tag scope: ASMBUS_Environment_Traffic_FellowMovement=global
  wires:
  In/1 -> [ASMBUS_Environment_Traffic_FellowMovement]
  [ASMBUS_Environment_Traffic_FellowMovement] -> Terminator_2/1

== system ASM_Traffic_MultiCore/Environment/Traffic/UserInterface/DISP_Plant ==
  In : Inport
  Bus Selector5 : BusSelector  OutputSignals=Traffic_Signals_toEnvironment.Info.TrafficState[]
  Fellow_Movement : Subsystem
  TrafficState[] : Subsystem
      mask Display: disp('')
  Traffic_State : Scope
      settings: TimeSpan=5  ActiveDisplayYMinimum=0.75  ActiveDisplayYMaximum=3.25  DataLoggingMaxPoints=20000  DataLoggingDecimation=10
  wires:
  In/1 -> Bus Selector5/1, Fellow_Movement/1(TrafficBus)
  Bus Selector5/1 -> TrafficState[]/1(In1)  "<TrafficState[]>"
  TrafficState[]/1(Out1) -> Traffic_State/1  "TrafficState[]"

== system ASM_Traffic_MultiCore/Environment/Traffic/UserInterface/PAR_Plant ==
  Bus Creator1 : BusCreator  Inputs=4
  Fellow_Doors : Subsystem
      mask Display: disp('Fellow Vehicle Doors')
  Fellow_VehicleLights : Subsystem
      mask Display: disp('Fellow Vehicle Lights')
  TrafficControl : Subsystem
      mask Display: disp('Traffic Control')
  V2X : Subsystem
      mask Display: disp('V2X')
  Out : Outport  VectorParamsAs1DForOutWhenUnconnected=off
  wires:
  Fellow_VehicleLights/1(Out1) -> Bus Creator1/2
  Bus Creator1/1 -> Out/1  "UserInterface"
  TrafficControl/1(Out1) -> Bus Creator1/1
  V2X/1(Out1) -> Bus Creator1/4
  Fellow_Doors/1(Out1) -> Bus Creator1/3

== system ASM_Traffic_MultiCore/VehicleDynamics/Control/SoftECU_Brake/Brake_Topology_Switch ==
  Enable_Trq_Brake_Extern[0|1] : Inport
  Trq_Brake_Request_Extern[Nm] : Inport  Port=2
  Trq_Request_Brake[Nm] : Inport  Port=3
  Vehicle_Topology[-2|-1|0|2] : Inport  Port=4
  Compare To Constant : simulink/Logic and Bit Operations/Compare To Constant  relop===  const=2  OutDataTypeStr=boolean
  Compare To Constant1 : simulink/Logic and Bit Operations/Compare To Constant  relop===  const=-2  OutDataTypeStr=boolean
  Constant : Constant
  OR : Logic  Operator=OR  AllPortsSameDT=off  OutDataTypeStr=boolean
  Switch : Switch  Criteria=u2 ~= 0  SaturateOnIntegerOverflow=off  InputSameDT=off
  Switch1 : Switch  Criteria=u2 ~= 0  SaturateOnIntegerOverflow=off  InputSameDT=off
  Enable_Trq_Extern[0|1] : Outport  VectorParamsAs1DForOutWhenUnconnected=off
  Trq_Request_Extern[Nm] : Outport  Port=2  VectorParamsAs1DForOutWhenUnconnected=off
  wires:
  Vehicle_Topology[-2|-1|0|2]/1 -> Compare To Constant1/1, Compare To Constant/1
  Constant/1 -> Switch/1
  Trq_Request_Brake[Nm]/1 -> Switch1/1
  Trq_Brake_Request_Extern[Nm]/1 -> Switch1/3
  Enable_Trq_Brake_Extern[0|1]/1 -> Switch/3
  Switch/1 -> Enable_Trq_Extern[0|1]/1
  Switch1/1 -> Trq_Request_Extern[Nm]/1
  OR/1 -> Switch1/2, Switch/2
  Compare To Constant/1 -> OR/1
  Compare To Constant1/1 -> OR/2

== system ASM_Traffic_MultiCore/VehicleDynamics/Control/SoftECU_Brake/Engine_Topology_Switch ==
  Vehicle_Topology[-2|-1|0|2] : Inport
  Trq_Eff_Engine[Nm] : Inport  Port=2
  Trq_EM_Front[Nm] : Inport  Port=3
  Compare To Constant : simulink/Logic and Bit Operations/Compare To Constant  relop===  const=-2  OutDataTypeStr=boolean
  Switch : Switch  Criteria=u2 ~= 0  SaturateOnIntegerOverflow=off  InputSameDT=off
  Trq[Nm] : Outport  VectorParamsAs1DForOutWhenUnconnected=off
  wires:
  Switch/1 -> Trq[Nm]/1
  Trq_EM_Front[Nm]/1 -> Switch/1
  Compare To Constant/1 -> Switch/2
  Trq_Eff_Engine[Nm]/1 -> Switch/3
  Vehicle_Topology[-2|-1|0|2]/1 -> Compare To Constant/1

== system ASM_Traffic_MultiCore/VehicleDynamics/Control/SoftECU_Brake/Map_Inputs ==
  Reset[0|1] : Inport
  Switches_ESP_User : Inport  Port=2
  ECU_Commands[] : Inport  Port=3
  Bus Selector2 : BusSelector  OutputSignals=Sw_ESP_Control_Mode[1ManSched|2Manual],Sw_ESP[0Off|1ABS|2ESP],Sw_ASR[0Off|1On]
  Maneuver : Subsystem
  Multiport Switch6 : MultiPortSwitch  Inputs=2  InputSameDT=off
  Multiport Switch7 : MultiPortSwitch  Inputs=2  InputSameDT=off
  Sw_ESP[0Off|1ABS|ESP] : Outport  VectorParamsAs1DForOutWhenUnconnected=off
  Sw_ASR[0Off|1On] : Outport  Port=2  VectorParamsAs1DForOutWhenUnconnected=off
  wires:
  Multiport Switch7/1 -> Sw_ESP[0Off|1ABS|ESP]/1
  Multiport Switch6/1 -> Sw_ASR[0Off|1On]/1
  Switches_ESP_User/1 -> Bus Selector2/1
  ECU_Commands[]/1 -> Maneuver/1(ECU_Commands[])
  Bus Selector2/1 -> Multiport Switch7/1, Multiport Switch6/1  "<Sw_ESP_Control_Mode[1ManSched|2Manual]>"
  Bus Selector2/2 -> Multiport Switch7/3  "<Sw_ESP[0Off|1ABS|2ESP]>"
  Bus Selector2/3 -> Multiport Switch6/3  "<Sw_ASR[0Off|1On]>"
  Maneuver/1(Sw_ESP[0Off|1ABS|2ESP]) -> Multiport Switch7/2
  Maneuver/2(Sw_ASR0Off|1On]) -> Multiport Switch6/2
  Reset[0|1]/1 -> Maneuver/2(Reset[0|1])

== system ASM_Traffic_MultiCore/VehicleDynamics/Control/SoftECU_Brake/Soft_ECU_Brake ==
  State_Brake_Without_BrkPedal[0|1] : Inport
  Enable_Trq_Extern[0|1] : Inport  Port=2
  Trq_Request_Extern[Nm] : Inport  Port=3
  Const_BrakeDiscFactor[FL;FR;RL;RR][m3] : Inport  Port=4
  Reset[] : Inport  Port=5
  Sw_ESP[0Off|1ABS|2ESP] : Inport  Port=6
  Sw_ASR[0Off|1On] : Inport  Port=7
  Trq_Eff_Engine[Nm] : Inport  Port=8
  p_MasterBrakeCyl[bar] : Inport  Port=9
  v_x_Vehicle_CoG[km|h] : Inport  Port=10
  v_y_Vehicle_CoG[km|h] : Inport  Port=11
  a_y_Vehicle_CoG[m|s2] : Inport  Port=12
  YawRate_Vehicle_CoG[deg|s] : Inport  Port=13
  WheelSpeed[FL;FR;RL;RR][rad|s] : Inport  Port=14
  Angle_SteeringWheel[deg] : Inport  Port=15
  i_Steering_Mean[] : Inport  Port=16
  Pos_AccPedal[%] : Inport  Port=17
  Pos_BrakePedal[%] : Inport  Port=18
  Pos_RL_Wheel[x;y;z][m] : Inport  Port=19
  Pos_FL_Wheel[x;y;z][m] : Inport  Port=20
  r_Tire[m] : Inport  Port=21
  ASMSignalCollector : Subsystem
  Bus Creator5 : BusCreator  Inputs=6
  Bus Creator6 : BusCreator  Inputs=13
  Bus2Vec : BusToVector
  Constant{1..20} (20 alike) : Constant  Value=0
  DESIRED_BRAKE_PRESSURE : ASM_BrakeHydraulics_lib/SoftECU/DESIRED_BRAKE_PRESSURE  Tag=ASM_SUBCOMPONENT  ASMProperties=struct('Name','DESIRED_BRAKE_PRESSURE','Version','2.0','Library','ASM_BrakeHydraulics_lib')  ASMInstanceName=desired_brake_pressure  ASMInstanceID=1
  Sum of Elements : Sum  Inputs=+
  Terminator_{1..18} (18 alike) : Terminator
  avoid_incomplete_trace2source : Subsystem
  ASMSignalBus : Outport  VectorParamsAs1DForOutWhenUnconnected=off
  Enable_p_Brake_Desired[0|1] : Outport  Port=2  VectorParamsAs1DForOutWhenUnconnected=off
  p_Brake_Desired[bar] : Outport  Port=3  VectorParamsAs1DForOutWhenUnconnected=off
  ECU_Mode[0None|1ABS|2ESP|3ASR] : Outport  Port=4  VectorParamsAs1DForOutWhenUnconnected=off
  Valves : Outport  Port=5  VectorParamsAs1DForOutWhenUnconnected=off
  Trq_Intervention : Outport  Port=6  VectorParamsAs1DForOutWhenUnconnected=off
  tag scope: ASMBUS_SoftECU_BrakeDesired=global
  wires:
  avoid_incomplete_trace2source/1(Out1) -> DESIRED_BRAKE_PRESSURE/1
  Enable_Trq_Extern[0|1]/1 -> avoid_incomplete_trace2source/1(In1)
  Sum of Elements/1 -> DESIRED_BRAKE_PRESSURE/3
  DESIRED_BRAKE_PRESSURE/1 -> [ASMBUS_SoftECU_BrakeDesired]
  Constant15/1 -> Bus Creator5/1  "Enable_TrqDecrease_Fast_ESP[0|1]"
  Constant17/1 -> Bus Creator5/3  "Enable_TrqDecrease_Slow_ESP[0|1]"
  Constant18/1 -> Bus Creator5/4  "Trq_DecreaseRequest_Slow_ESP[Nm]"
  Constant5/1 -> Bus Creator5/5  "Enable_TrqIncrease_ESP[0|1]"
  Constant6/1 -> Bus Creator5/6  "Trq_IncreaseRequest_ESP[Nm]"
  Constant7/1 -> Bus Creator6/6  "Ctrl_InletValve_FL[0_1]"
  Constant8/1 -> Bus Creator6/7  "Ctrl_InletValve_FR[0_1]"
  Constant9/1 -> Bus Creator6/8  "Ctrl_InletValve_RL[0_1]"
  Constant10/1 -> Bus Creator6/9  "Ctrl_InletValve_RR[0_1]"
  Constant11/1 -> Bus Creator6/10  "Ctrl_OutletValve_FL[0_1]"
  Constant12/1 -> Bus Creator6/11  "Ctrl_OutletValve_FR[0_1]"
  Constant13/1 -> Bus Creator6/12  "Ctrl_OutletValve_RL[0_1]"
  Constant14/1 -> Bus Creator6/13  "Ctrl_OutletValve_RR[0_1]"
  Constant1/1 -> Bus Creator6/2  "Ctrl_PreChargeValve_1[0_1]"
  Constant2/1 -> Bus Creator6/3  "Ctrl_PreChargeValve_2[0_1]"
  Constant3/1 -> Bus Creator6/4  "Ctrl_ChangeOverValve_1[0_1]"
  Constant4/1 -> Bus Creator6/5  "Ctrl_ChangeOverValve_2[0_1]"
  DESIRED_BRAKE_PRESSURE/2 -> Enable_p_Brake_Desired[0|1]/1  "Enable_p_Brake_Desired[0|1]"
  DESIRED_BRAKE_PRESSURE/3 -> p_Brake_Desired[bar]/1  "p_Brake_Desired[bar]"
  Bus Creator5/1 -> Trq_Intervention/1  "Trq_Intervention"
  Trq_Request_Extern[Nm]/1 -> DESIRED_BRAKE_PRESSURE/2
  Bus Creator6/1 -> Valves/1  "Valves"
  Const_BrakeDiscFactor[FL;FR;RL;RR][m3]/1 -> Bus2Vec/1
  Bus2Vec/1 -> Sum of Elements/1
  Constant16/1 -> Bus Creator5/2  "Trq_DecreaseRequest_Fast_ESP[Nm]"
  Constant19/1 -> Bus Creator6/1  "Ctrl_HydPump[0_1]"
  Constant20/1 -> ECU_Mode[0None|1ABS|2ESP|3ASR]/1  "ECU_Mode[0None|1ABS|2ESP|3ASR]"
  Reset[]/1 -> Terminator_1/1
  Sw_ESP[0Off|1ABS|2ESP]/1 -> Terminator_2/1
  Sw_ASR[0Off|1On]/1 -> Terminator_3/1
  Trq_Eff_Engine[Nm]/1 -> Terminator_4/1
  p_MasterBrakeCyl[bar]/1 -> Terminator_5/1
  v_x_Vehicle_CoG[km|h]/1 -> Terminator_6/1
  v_y_Vehicle_CoG[km|h]/1 -> Terminator_7/1
  a_y_Vehicle_CoG[m|s2]/1 -> Terminator_8/1
  YawRate_Vehicle_CoG[deg|s]/1 -> Terminator_9/1
  WheelSpeed[FL;FR;RL;RR][rad|s]/1 -> Terminator_10/1
  Angle_SteeringWheel[deg]/1 -> Terminator_11/1
  i_Steering_Mean[]/1 -> Terminator_12/1
  Pos_AccPedal[%]/1 -> Terminator_13/1
  Pos_BrakePedal[%]/1 -> Terminator_14/1
  Pos_RL_Wheel[x;y;z][m]/1 -> Terminator_15/1
  Pos_FL_Wheel[x;y;z][m]/1 -> Terminator_16/1
  r_Tire[m]/1 -> Terminator_17/1
  ASMSignalCollector/1(ASMSignalBus) -> ASMSignalBus/1
  State_Brake_Without_BrkPedal[0|1]/1 -> Terminator_18/1

== system ASM_Traffic_MultiCore/VehicleDynamics/Control/Sw_ECU_Brake_Signals/Ctrl_ChangeOverValve_1[0_1] ==
  SoftECU : Inport
  RealECU : Inport  Port=2
  Const_Ctrl_ChangeOverValve_1[0_1] : Constant  Value=0
  MultiPortSwitch : MultiPortSwitch
  Sw_Ctrl_ChangeOverValve_1[1SoftECU|2RealECU|3Const] : Constant  Value=CPT.MDL_SW.Sw_Ctrl_ChangeOverValve_1.v
  Ctrl_ChangeOverValve_1[0_1] : Outport  VectorParamsAs1DForOutWhenUnconnected=off
  wires:
  MultiPortSwitch/1 -> Ctrl_ChangeOverValve_1[0_1]/1
  Const_Ctrl_ChangeOverValve_1[0_1]/1 -> MultiPortSwitch/4
  RealECU/1 -> MultiPortSwitch/3
  SoftECU/1 -> MultiPortSwitch/2
  Sw_Ctrl_ChangeOverValve_1[1SoftECU|2RealECU|3Const]/1 -> MultiPortSwitch/1

== system ASM_Traffic_MultiCore/VehicleDynamics/Control/Sw_ECU_Brake_Signals/Ctrl_ChangeOverValve_2[0_1] ==
  SoftECU : Inport
  RealECU : Inport  Port=2
  Const_Ctrl_ChangeOverValve_2[0_1] : Constant  Value=0
  MultiPortSwitch : MultiPortSwitch
  Sw_Ctrl_ChangeOverValve_2[1SoftECU|2RealECU|3Const] : Constant  Value=CPT.MDL_SW.Sw_Ctrl_ChangeOverValve_2.v
  Ctrl_ChangeOverValve_2[0_1] : Outport  VectorParamsAs1DForOutWhenUnconnected=off
  wires:
  Sw_Ctrl_ChangeOverValve_2[1SoftECU|2RealECU|3Const]/1 -> MultiPortSwitch/1
  SoftECU/1 -> MultiPortSwitch/2
  RealECU/1 -> MultiPortSwitch/3
  Const_Ctrl_ChangeOverValve_2[0_1]/1 -> MultiPortSwitch/4
  MultiPortSwitch/1 -> Ctrl_ChangeOverValve_2[0_1]/1

== system ASM_Traffic_MultiCore/VehicleDynamics/Control/Sw_ECU_Brake_Signals/Ctrl_HydPump[0_1] ==
  SoftECU : Inport
  RealECU : Inport  Port=2
  Const_Ctrl_HydPump[0_1] : Constant  Value=0
  MultiPortSwitch : MultiPortSwitch
  Sw_Ctrl_HydPump[1SoftECU|2RealECU|3Const] : Constant  Value=CPT.MDL_SW.Sw_Ctrl_HydPump.v
  Ctrl_HydPump[0_1] : Outport  VectorParamsAs1DForOutWhenUnconnected=off
  wires:
  Sw_Ctrl_HydPump[1SoftECU|2RealECU|3Const]/1 -> MultiPortSwitch/1
  SoftECU/1 -> MultiPortSwitch/2
  RealECU/1 -> MultiPortSwitch/3
  Const_Ctrl_HydPump[0_1]/1 -> MultiPortSwitch/4
  MultiPortSwitch/1 -> Ctrl_HydPump[0_1]/1

== system ASM_Traffic_MultiCore/VehicleDynamics/Control/Sw_ECU_Brake_Signals/Ctrl_InletValve_FL[0_1] ==
  SoftECU : Inport
  RealECU : Inport  Port=2
  Const_Ctrl_InletValve_FL[0_1] : Constant  Value=0
  MultiPortSwitch : MultiPortSwitch
  Sw_Ctrl_InletValve_FL[1SoftECU|2RealECU|3Const] : Constant  Value=CPT.MDL_SW.Sw_Ctrl_InletValve_FL.v
  Ctrl_InletValve_FL[0_1] : Outport  VectorParamsAs1DForOutWhenUnconnected=off
  wires:
  Sw_Ctrl_InletValve_FL[1SoftECU|2RealECU|3Const]/1 -> MultiPortSwitch/1
  SoftECU/1 -> MultiPortSwitch/2
  RealECU/1 -> MultiPortSwitch/3
  Const_Ctrl_InletValve_FL[0_1]/1 -> MultiPortSwitch/4
  MultiPortSwitch/1 -> Ctrl_InletValve_FL[0_1]/1

== system ASM_Traffic_MultiCore/VehicleDynamics/Control/Sw_ECU_Brake_Signals/Ctrl_InletValve_FR[0_1] ==
  SoftECU : Inport
  RealECU : Inport  Port=2
  Const_Ctrl_InletValve_FR[0_1] : Constant  Value=0
  MultiPortSwitch : MultiPortSwitch
  Sw_Ctrl_InletValve_FR[1SoftECU|2RealECU|3Const] : Constant  Value=CPT.MDL_SW.Sw_Ctrl_InletValve_FR.v
  Ctrl_InletValve_FR[0_1] : Outport  VectorParamsAs1DForOutWhenUnconnected=off
  wires:
  MultiPortSwitch/1 -> Ctrl_InletValve_FR[0_1]/1
  Const_Ctrl_InletValve_FR[0_1]/1 -> MultiPortSwitch/4
  RealECU/1 -> MultiPortSwitch/3
  SoftECU/1 -> MultiPortSwitch/2
  Sw_Ctrl_InletValve_FR[1SoftECU|2RealECU|3Const]/1 -> MultiPortSwitch/1

== system ASM_Traffic_MultiCore/VehicleDynamics/Control/Sw_ECU_Brake_Signals/Ctrl_InletValve_RL[0_1] ==
  SoftECU : Inport
  RealECU : Inport  Port=2
  Const_Ctrl_InletValve_RL[0_1] : Constant  Value=0
  MultiPortSwitch : MultiPortSwitch
  Sw_Ctrl_InletValve_RL[1SoftECU|2RealECU|3Const] : Constant  Value=CPT.MDL_SW.Sw_Ctrl_InletValve_RL.v
  Ctrl_InletValve_RL[0_1] : Outport  VectorParamsAs1DForOutWhenUnconnected=off
  wires:
  MultiPortSwitch/1 -> Ctrl_InletValve_RL[0_1]/1
  Const_Ctrl_InletValve_RL[0_1]/1 -> MultiPortSwitch/4
  RealECU/1 -> MultiPortSwitch/3
  SoftECU/1 -> MultiPortSwitch/2
  Sw_Ctrl_InletValve_RL[1SoftECU|2RealECU|3Const]/1 -> MultiPortSwitch/1

== system ASM_Traffic_MultiCore/VehicleDynamics/Control/Sw_ECU_Brake_Signals/Ctrl_InletValve_RR[0_1] ==
  SoftECU : Inport
  RealECU : Inport  Port=2
  Const_Ctrl_InletValve_RR[0_1] : Constant  Value=0
  MultiPortSwitch : MultiPortSwitch
  Sw_Ctrl_InletValve_RR[1SoftECU|2RealECU|3Const] : Constant  Value=CPT.MDL_SW.Sw_Ctrl_InletValve_RR.v
  Ctrl_InletValve_RR[0_1] : Outport  VectorParamsAs1DForOutWhenUnconnected=off
  wires:
  Sw_Ctrl_InletValve_RR[1SoftECU|2RealECU|3Const]/1 -> MultiPortSwitch/1
  SoftECU/1 -> MultiPortSwitch/2
  RealECU/1 -> MultiPortSwitch/3
  Const_Ctrl_InletValve_RR[0_1]/1 -> MultiPortSwitch/4
  MultiPortSwitch/1 -> Ctrl_InletValve_RR[0_1]/1

== system ASM_Traffic_MultiCore/VehicleDynamics/Control/Sw_ECU_Brake_Signals/Ctrl_OutletValve_FL[0_1] ==
  SoftECU : Inport
  RealECU : Inport  Port=2
  Const_Ctrl_OutletValve_FL[0_1] : Constant  Value=0
  MultiPortSwitch : MultiPortSwitch
  Sw_Ctrl_OutletValve_FL[1SoftECU|2RealECU|3Const] : Constant  Value=CPT.MDL_SW.Sw_Ctrl_OutletValve_FL.v
  Ctrl_OutletValve_FL[0_1] : Outport  VectorParamsAs1DForOutWhenUnconnected=off
  wires:
  Sw_Ctrl_OutletValve_FL[1SoftECU|2RealECU|3Const]/1 -> MultiPortSwitch/1
  SoftECU/1 -> MultiPortSwitch/2
  RealECU/1 -> MultiPortSwitch/3
  Const_Ctrl_OutletValve_FL[0_1]/1 -> MultiPortSwitch/4
  MultiPortSwitch/1 -> Ctrl_OutletValve_FL[0_1]/1

== system ASM_Traffic_MultiCore/VehicleDynamics/Control/Sw_ECU_Brake_Signals/Ctrl_OutletValve_FR[0_1] ==
  SoftECU : Inport
  RealECU : Inport  Port=2
  Const_Ctrl_OutletValve_FR[0_1] : Constant  Value=0
  MultiPortSwitch : MultiPortSwitch
  Sw_Ctrl_OutletValve_FR[1SoftECU|2RealECU|3Const] : Constant  Value=CPT.MDL_SW.Sw_Ctrl_OutletValve_FR.v
  Ctrl_OutletValve_FR[0_1] : Outport  VectorParamsAs1DForOutWhenUnconnected=off
  wires:
  MultiPortSwitch/1 -> Ctrl_OutletValve_FR[0_1]/1
  Const_Ctrl_OutletValve_FR[0_1]/1 -> MultiPortSwitch/4
  RealECU/1 -> MultiPortSwitch/3
  SoftECU/1 -> MultiPortSwitch/2
  Sw_Ctrl_OutletValve_FR[1SoftECU|2RealECU|3Const]/1 -> MultiPortSwitch/1

== system ASM_Traffic_MultiCore/VehicleDynamics/Control/Sw_ECU_Brake_Signals/Ctrl_OutletValve_RL[0_1] ==
  SoftECU : Inport
  RealECU : Inport  Port=2
  Const_Ctrl_OutletValve_RL[0_1] : Constant  Value=0
  MultiPortSwitch : MultiPortSwitch
  Sw_Ctrl_OutletValve_RL[1SoftECU|2RealECU|3Const] : Constant  Value=CPT.MDL_SW.Sw_Ctrl_OutletValve_RL.v
  Ctrl_OutletValve_RL[0_1] : Outport  VectorParamsAs1DForOutWhenUnconnected=off
  wires:
  MultiPortSwitch/1 -> Ctrl_OutletValve_RL[0_1]/1
  Const_Ctrl_OutletValve_RL[0_1]/1 -> MultiPortSwitch/4
  RealECU/1 -> MultiPortSwitch/3
  SoftECU/1 -> MultiPortSwitch/2
  Sw_Ctrl_OutletValve_RL[1SoftECU|2RealECU|3Const]/1 -> MultiPortSwitch/1

== system ASM_Traffic_MultiCore/VehicleDynamics/Control/Sw_ECU_Brake_Signals/Ctrl_OutletValve_RR[0_1] ==
  SoftECU : Inport
  RealECU : Inport  Port=2
  Const_Ctrl_OutletValve_RR[0_1] : Constant  Value=0
  MultiPortSwitch : MultiPortSwitch
  Sw_Ctrl_OutletValve_RR[1SoftECU|2RealECU|3Const] : Constant  Value=CPT.MDL_SW.Sw_Ctrl_OutletValve_RR.v
  Ctrl_OutletValve_RR[0_1] : Outport  VectorParamsAs1DForOutWhenUnconnected=off
  wires:
  Sw_Ctrl_OutletValve_RR[1SoftECU|2RealECU|3Const]/1 -> MultiPortSwitch/1
  SoftECU/1 -> MultiPortSwitch/2
  RealECU/1 -> MultiPortSwitch/3
  Const_Ctrl_OutletValve_RR[0_1]/1 -> MultiPortSwitch/4
  MultiPortSwitch/1 -> Ctrl_OutletValve_RR[0_1]/1

== system ASM_Traffic_MultiCore/VehicleDynamics/Control/Sw_ECU_Brake_Signals/Ctrl_PreChargeValve_1[0_1] ==
  SoftECU : Inport
  RealECU : Inport  Port=2
  Const_Ctrl_PreChargeValve_1[0_1] : Constant  Value=0
  MultiPortSwitch : MultiPortSwitch
  Sw_Ctrl_PreChargeValve_1[1SoftECU|2RealECU|3Const] : Constant  Value=CPT.MDL_SW.Sw_Ctrl_PreChargeValve_1.v
  Ctrl_PreChargeValve_1[0_1] : Outport  VectorParamsAs1DForOutWhenUnconnected=off
  wires:
  Sw_Ctrl_PreChargeValve_1[1SoftECU|2RealECU|3Const]/1 -> MultiPortSwitch/1
  SoftECU/1 -> MultiPortSwitch/2
  RealECU/1 -> MultiPortSwitch/3
  Const_Ctrl_PreChargeValve_1[0_1]/1 -> MultiPortSwitch/4
  MultiPortSwitch/1 -> Ctrl_PreChargeValve_1[0_1]/1

== system ASM_Traffic_MultiCore/VehicleDynamics/Control/Sw_ECU_Brake_Signals/Ctrl_PreChargeValve_2[0_1] ==
  SoftECU : Inport
  RealECU : Inport  Port=2
  Const_Ctrl_PreChargeValve_2[0_1] : Constant  Value=0
  MultiPortSwitch : MultiPortSwitch
  Sw_Ctrl_PreChargeValve_2[1SoftECU|2RealECU|3Const] : Constant  Value=CPT.MDL_SW.Sw_Ctrl_PreChargeValve_2.v
  Ctrl_PreChargeValve_2[0_1] : Outport  VectorParamsAs1DForOutWhenUnconnected=off
  wires:
  MultiPortSwitch/1 -> Ctrl_PreChargeValve_2[0_1]/1
  Const_Ctrl_PreChargeValve_2[0_1]/1 -> MultiPortSwitch/4
  RealECU/1 -> MultiPortSwitch/3
  SoftECU/1 -> MultiPortSwitch/2
  Sw_Ctrl_PreChargeValve_2[1SoftECU|2RealECU|3Const]/1 -> MultiPortSwitch/1

== system ASM_Traffic_MultiCore/VehicleDynamics/Control/Sw_ECU_Brake_Signals/ECU_ESP_Mode[0None|1ABS|2ESP|3ASR] ==
  SoftECU : Inport
  RealECU : Inport  Port=2
  Const_ECU_ESP_Mode[0None|1ABS|2ESP|3ASR] : Constant  Value=0
  MultiPortSwitch : MultiPortSwitch
  Sw_ECU_Mode[1SoftECU|2RealECU|3Const] : Constant  Value=CPT.MDL_SW.Sw_ECU_ESP_Mode.v
  ECU_ESP_Mode[0None|1ABS|2ESP|3ASR] : Outport  VectorParamsAs1DForOutWhenUnconnected=off
  wires:
  MultiPortSwitch/1 -> ECU_ESP_Mode[0None|1ABS|2ESP|3ASR]/1
  Const_ECU_ESP_Mode[0None|1ABS|2ESP|3ASR]/1 -> MultiPortSwitch/4
  RealECU/1 -> MultiPortSwitch/3
  SoftECU/1 -> MultiPortSwitch/2
  Sw_ECU_Mode[1SoftECU|2RealECU|3Const]/1 -> MultiPortSwitch/1
